simulink model "compare_lin"  (R2026b)
settings: Solver=VariableStepAuto  StopTime=15
PostLoadFcn:
  | run(fullfile(fileparts(get_param(bdroot, 'FileName')), 'parameters.m'));
InitFcn:
  | run(fullfile(fileparts(get_param(bdroot, 'FileName')), 'parameters.m'));
values from neighbouring files (symbols this model uses):
  dWf = 0.748    [parameters.m]
  k = 50    [parameters.m]
  K = 1/a    [make_figures.m]    (also in parameters.m)
  n = 2.7    [parameters.m]
  N0 = cases{i,1}    [make_figures.m]
  tau = 1/(P.k*a)    [make_figures.m]    (also in parameters.m = 1/(k*a))
  Wf0 = (N0/100)^P.n    [make_figures.m]    (also in parameters.m = (N0/100)^n; run_lin.m = (N0/100)^n)
settings Model: Creator=a  LastModifiedBy=a

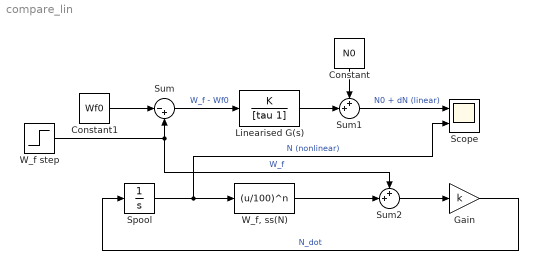
== system compare_lin ==
  Constant : Constant  Value=N0
  Constant1 : Constant  Value=Wf0
  Gain : Gain  Gain=k
  Linearised G(s) : TransferFcn  Numerator=K  Denominator=[tau 1]
  Scope : Scope  NumInputPorts=2
      settings: ActiveDisplayYMinimum=22.996227382080747  ActiveDisplayYMaximum=144.06892767650712
  Spool : Integrator  InitialCondition=N0
  Sum : Sum  Inputs=|-+
  Sum1 : Sum  Inputs=++|
  Sum2 : Sum  Inputs=++|
  W_f step : Step  Time=2  InitialValue=Wf0  FinalValue=Wf0 + dWf  SampleTime=0
  "W_f, ss(N)" : Fcn  Expr=(u/100)^n
  wires:
  Spool/1 -> Scope/2, "W_f, ss(N)"/1  "N (nonlinear)"
  "W_f, ss(N)"/1 -> Sum2/2
  Sum2/1 -> Gain/1
  Gain/1 -> Spool/1  "N_dot"
  W_f step/1 -> Sum2/1, Sum/2  "W_f"
  Linearised G(s)/1 -> Sum1/2
  Constant/1 -> Sum1/1
  Constant1/1 -> Sum/1
  Sum/1 -> Linearised G(s)/1  "W_f - Wf0"
  Sum1/1 -> Scope/1  "N0 + dN (linear)"
